simulink model "anc_system"  (R2025b)
settings: Solver=ode23  StartTime=0.0  StopTime=37  FixedStep=256/44100  RelTol=1e-3
libraries: fl_lib x25, ee_lib x5, nesl_utility x4, dspvision x1
settings Model: Creator=Asus  LastModifiedBy=asus
settings SolverCC: ZeroCrossAlgorithm=Adaptive
settings DebuggingCC: MaskedZcDiagnostic=none  IgnoredZcDiagnostic=none

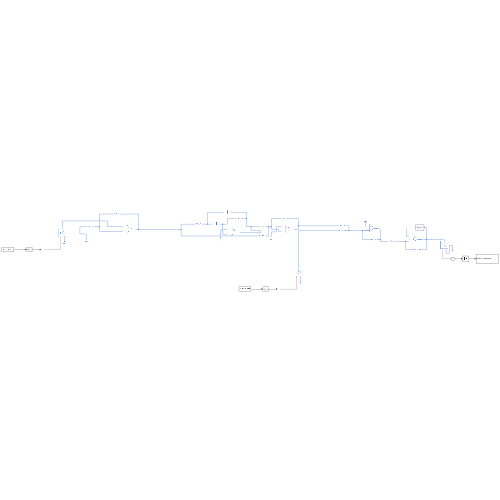
[thumbnail: Simulink's stored preview of the top-level diagram]
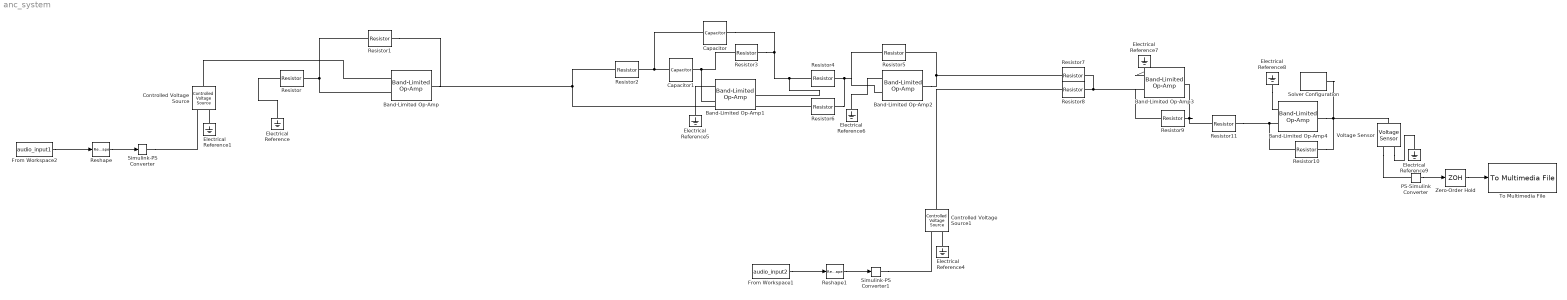
== system anc_system ==
  Band-Limited Op-Amp{,1..4} (5 alike) : ee_lib/Integrated Circuits/Band-Limited Op-Amp  A=200000  Rin=50e6 Ohm  Rout=60 Ohm  Vmin=-15 V  Vmax=15 V  Vdotmax=300000 V/s  f=6e5 Hz  V0=0 V
  Capacitor : fl_lib/Electrical/Electrical Elements/Capacitor  c=10 nF  r=1e-6 Ohm  g=0 1/Ohm  i_specify=off  i_priority=None  i=0 A  i_nominal_specify=off  i_nominal_value=1  i_nominal_unit=A  v_specify=off  v_priority=None  v=0 V  v_nominal_specify=off  v_nominal_value=1  v_nominal_unit=V  vc_specify=off  vc_priority=High  vc=0 V  vc_nominal_specify=off  vc_nominal_value=1  vc_nominal_unit=V
  Capacitor1 : fl_lib/Electrical/Electrical Elements/Capacitor  c=10 nF  r=1e-6 Ohm  g=0 1/Ohm  i_specify=off  i_priority=None  i=0 A  i_nominal_specify=off  i_nominal_value=1  i_nominal_unit=A  v_specify=off  v_priority=None  v=0 V  v_nominal_specify=off  v_nominal_value=1  v_nominal_unit=V  vc_specify=off  vc_priority=High  vc=0 V  vc_nominal_specify=off  vc_nominal_value=1  vc_nominal_unit=V
  Controlled Voltage Source : fl_lib/Electrical/Electrical Sources/Controlled Voltage Source
  Controlled Voltage Source1 : fl_lib/Electrical/Electrical Sources/Controlled Voltage Source
  Electrical Reference{,1,4..9} (8 alike) : fl_lib/Electrical/Electrical Elements/Electrical Reference
  From Workspace1 : FromWorkspace  VariableName=audio_input2  SampleTime=1/44100
  From Workspace2 : FromWorkspace  VariableName=audio_input1  SampleTime=1/44100
  PS-Simulink Converter : nesl_utility/PS-Simulink Converter  PhysicalDomain=network_engine_domain  SubClassName=ps_output  LeftPortType=input  RightPortType=output  PseudoPeriodic=off  Frequencies=[]  VectorFormat=inherit  Unit=inherit  AffineConversion=off
  Reshape : Reshape
  Reshape1 : Reshape
  Resistor{,7..11} (6 alike) : fl_lib/Electrical/Electrical Elements/Resistor  R=1 kOhm  i_specify=off  i_priority=None  i=0 A  i_nominal_specify=off  i_nominal_value=1  i_nominal_unit=A  v_specify=off  v_priority=None  v=0 V  v_nominal_specify=off  v_nominal_value=1  v_nominal_unit=V
  Resistor1 : fl_lib/Electrical/Electrical Elements/Resistor  R=9 kOhm  i_specify=off  i_priority=None  i=0 A  i_nominal_specify=off  i_nominal_value=1  i_nominal_unit=A  v_specify=off  v_priority=None  v=0 V  v_nominal_specify=off  v_nominal_value=1  v_nominal_unit=V
  Resistor2 : fl_lib/Electrical/Electrical Elements/Resistor  R=1.25 kOhm  i_specify=off  i_priority=None  i=0 A  i_nominal_specify=off  i_nominal_value=1  i_nominal_unit=A  v_specify=off  v_priority=None  v=0 V  v_nominal_specify=off  v_nominal_value=1  v_nominal_unit=V
  Resistor3 : fl_lib/Electrical/Electrical Elements/Resistor  R=1.25 kOhm  i_specify=off  i_priority=None  i=0 A  i_nominal_specify=off  i_nominal_value=1  i_nominal_unit=A  v_specify=off  v_priority=None  v=0 V  v_nominal_specify=off  v_nominal_value=1  v_nominal_unit=V
  Resistor4 : fl_lib/Electrical/Electrical Elements/Resistor  R=1.12 kOhm  i_specify=off  i_priority=None  i=0 A  i_nominal_specify=off  i_nominal_value=1  i_nominal_unit=A  v_specify=off  v_priority=None  v=0 V  v_nominal_specify=off  v_nominal_value=1  v_nominal_unit=V
  Resistor5 : fl_lib/Electrical/Electrical Elements/Resistor  R=4 kOhm  i_specify=off  i_priority=None  i=0 A  i_nominal_specify=off  i_nominal_value=1  i_nominal_unit=A  v_specify=off  v_priority=None  v=0 V  v_nominal_specify=off  v_nominal_value=1  v_nominal_unit=V
  Resistor6 : fl_lib/Electrical/Electrical Elements/Resistor  R=4 kOhm  i_specify=off  i_priority=None  i=0 A  i_nominal_specify=off  i_nominal_value=1  i_nominal_unit=A  v_specify=off  v_priority=None  v=0 V  v_nominal_specify=off  v_nominal_value=1  v_nominal_unit=V
  Simulink-PS Converter : nesl_utility/Simulink-PS Converter  PhysicalDomain=network_engine_domain  SubClassName=ps_input  LeftPortType=input  RightPortType=output  PseudoPeriodic=off  Frequencies=[]  NoiseDistribution=none  NoiseParameters=[]  Unit=1  AffineConversion=off  FilteringAndDerivatives=provide  SimscapeFilterOrder=1  InputFilterTimeConstant=0.001  UdotUserProvided=0
  Simulink-PS Converter1 : nesl_utility/Simulink-PS Converter  PhysicalDomain=network_engine_domain  SubClassName=ps_input  LeftPortType=input  RightPortType=output  PseudoPeriodic=off  Frequencies=[]  NoiseDistribution=none  NoiseParameters=[]  Unit=1  AffineConversion=off  FilteringAndDerivatives=provide  SimscapeFilterOrder=1  InputFilterTimeConstant=0.001  UdotUserProvided=0
  Solver Configuration : nesl_utility/Solver Configuration  PhysicalDomain=network_engine_domain  SubClassName=solver  LeftPortType=input  RightPortType=generic  Tones=[]  Harmonics=[]  SimulateNoise=off  Profile=off  UseLocalSampling=off  EnableSwitchedLinearOptims=on  FrequencyDomain=off  UseCCode=off  RelTol=0.001  AbsTol=0.001  MinStep=1e-09  ToWorkspace=off  RevertToSquareIcSolve=off  NumHomotopyIterations=100  PhasorMode=off  PhasorModeNumHarmonics=1  ConsistencySolver=NEWTON_XTOL_AFTER_FTOL  IndexReductionMethod=DerivativeReplacement  DoDC=off  ResidualTolerance=1e-09  ConsistencyTolSource=GLOBAL  ConsistencyAbsTol=0.001  ConsistencyRelTol=0.001  ConsistencyTolFactor=0.001  UseLocalSolver=on  LocalSolverChoice=NE_BACKWARD_EULER_ADVANCER  ResolveIndetEquations=on  FunctionEvalNumThread=1  LocalSolverSampleTime=1/44100  DoFixedCost=off  MaxNonlinIter=3  MaxModeIter=2  ComputeImpulses=off  ImpulseIterations=2  LinearAlgebra=auto  LinearAlgebraNumThread=0  EquationFormulation=NE_TIME_EF  DelaysMemoryBudget=1024  AutomaticFiltering=on  FilteringTimeConstant=0.001  PartitionStorageMethod=AS_NEEDED  PartitionMemoryBudget=1024  PartitionMethod=ROBUST  MultibodyUseLocalSolver=off  MultibodyLocalSolverChoice=ODE1  MultibodyLocalSolverSampleTime=0.001
  To Multimedia File : dspvision/To Multimedia File  outputFilename=C:\Users\asus\OneDrive\Desktop\output.wav  streamSelection=Audio only  videoCompressor=None (uncompressed)  audioCompressor=None (uncompressed)  imagePorts=One multidimensional signal  fileType=WAV  audioDatatype=16-bit integer  fourcc=RGB  audioBitRate=128  audioQuality=75  videoQuality=75  mj2000CompFactor=10
      settings: LibrarySourceBlock=audiosinks/To Multimedia File
  Voltage Sensor : fl_lib/Electrical/Electrical Sensors/Voltage Sensor
  Zero-Order Hold : ZeroOrderHold  SampleTime=1/44100
  wires:
  From Workspace2/1 -> Reshape/1
  Reshape/1 -> Simulink-PS Converter/1
  From Workspace1/1 -> Reshape1/1
  Reshape1/1 -> Simulink-PS Converter1/1
  PS-Simulink Converter/1 -> Zero-Order Hold/1
  Zero-Order Hold/1 -> To Multimedia File/1
  connections:
  Resistor1/LConn1 -- Band-Limited Op-Amp/LConn2 -- Resistor/RConn1
  Resistor/LConn1 -- Electrical Reference/LConn1
  Simulink-PS Converter/RConn1 -- Controlled Voltage Source/RConn1
  Electrical Reference1/LConn1 -- Controlled Voltage Source/RConn2
  Capacitor/LConn1 -- Capacitor1/LConn1 -- Resistor2/RConn1
  Resistor2/LConn1 -- Resistor1/RConn1 -- Band-Limited Op-Amp/RConn1 -- Resistor6/LConn1
  Capacitor/RConn1 -- Resistor3/RConn1 -- Resistor4/LConn1 -- Band-Limited Op-Amp1/RConn1
  Electrical Reference4/LConn1 -- Controlled Voltage Source1/RConn2
  Simulink-PS Converter1/RConn1 -- Controlled Voltage Source1/RConn1
  Capacitor1/RConn1 -- Band-Limited Op-Amp1/LConn2 -- Resistor3/LConn1
  Resistor4/RConn1 -- Resistor5/LConn1 -- Band-Limited Op-Amp2/LConn2 -- Resistor6/RConn1
  Band-Limited Op-Amp2/RConn1 -- Resistor7/LConn1 -- Resistor5/RConn1
  Resistor8/RConn1 -- Resistor9/LConn1 -- Band-Limited Op-Amp3/LConn2 -- Resistor7/RConn1
  Band-Limited Op-Amp3/LConn1 -- Electrical Reference7/LConn1
  Resistor9/RConn1 -- Band-Limited Op-Amp3/RConn1 -- Resistor11/LConn1
  Resistor11/RConn1 -- Resistor10/LConn1 -- Band-Limited Op-Amp4/LConn2
  Electrical Reference8/LConn1 -- Band-Limited Op-Amp4/LConn1
  Band-Limited Op-Amp1/LConn1 -- Electrical Reference5/LConn1
  Electrical Reference6/LConn1 -- Band-Limited Op-Amp2/LConn1
  Band-Limited Op-Amp/LConn1 -- Controlled Voltage Source/LConn1
  Controlled Voltage Source1/LConn1 -- Resistor8/LConn1
  Band-Limited Op-Amp4/RConn1 -- Voltage Sensor/LConn1 -- Solver Configuration/RConn1 -- Resistor10/RConn1
  Voltage Sensor/RConn1 -- PS-Simulink Converter/LConn1
  Voltage Sensor/RConn2 -- Electrical Reference9/LConn1
